simulink model "Three_VSC_Microgrid_Droop_Control"  (R2025a)
settings: Solver=VariableStepAuto  StartTime=0.0  StopTime=10  RelTol=1e-3
InitFcn:
  | fsw=10e3;
  | fref=50;
  | Ts=1/(fsw*fref);
  | Vodref=220*sqrt(2);
  | Voqref=0;
  | Vdc=700;
  | w0=2*pi*fref;
  | 
  | Lf=3.5e-3;
  | Rf=0.1;
  | Cf=50e-6;
  | Lc=0.35e-3;
  | Rc=0.05;
  | 
  | Tci=4/(2*pi*fsw);
  | wci=1/Tci;
  | Kpc=Lf*wci;
  | Kic=Rf*wci;
  | 
  | pm=50;
  | wcv=1/Tci*(1-sind(pm))/(1+sind(pm));
  | wgc=sqrt(wcv*wci);
  | Kpv=Cf*wgc;
  | Kiv=Kpv*wcv;
  | 
  | mp=5e-5;
  | np=3e-3;
libraries: spsThreePhaseSeriesRLCBranchLib x12, slpidlib x12, spsabctodq0Lib x9, spsThreePhaseVIMeasurementLib x6, spsThreePhaseSeriesRLCLoadLib x4, spsDCVoltageSourceLib x3, spsGroundLib x3, spsPWMGenerator2LevelLib x3, spsUniversalBridgeLib x3, spsdq0toabcLib x3, spsThreePhaseBreakerLib x1, spspowerguiLib x1
(part 1 of 2)
settings Model: Creator=DELL  LastModifiedBy=bhargabgogoi

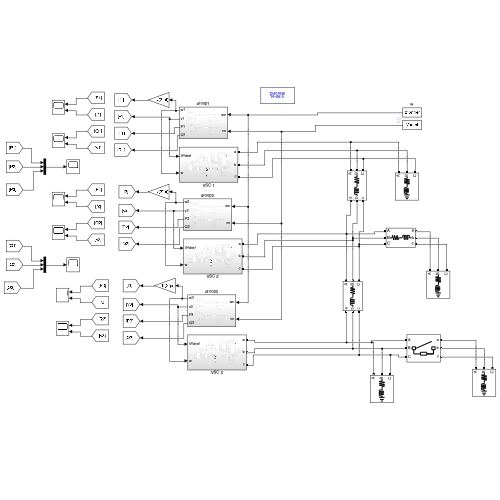
[thumbnail: Simulink's stored preview of the top-level diagram]
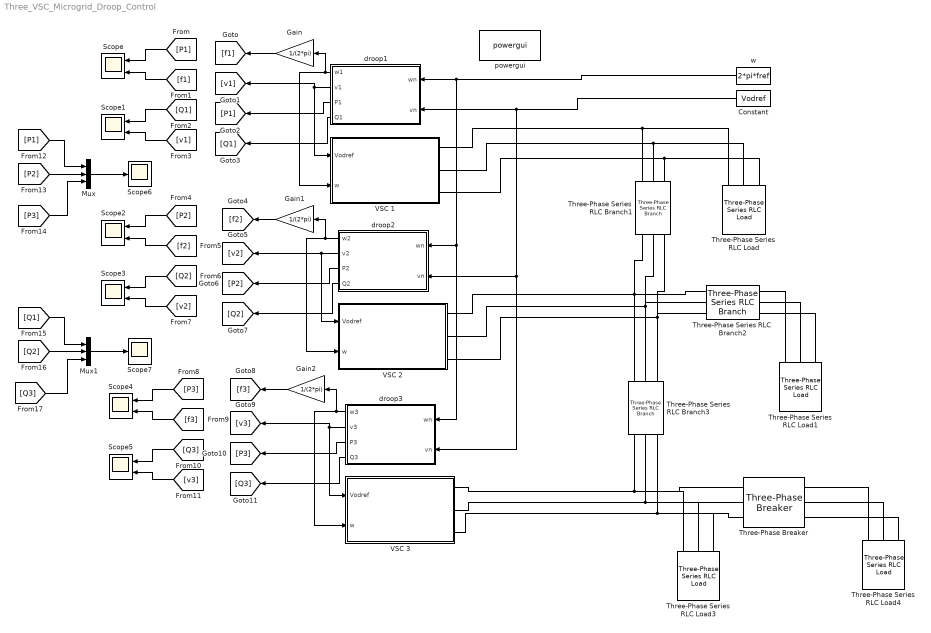
== system Three_VSC_Microgrid_Droop_Control ==
  Constant : Constant  Value=Vodref
  Gain : Gain  Gain=1/(2*pi)
  Gain1 : Gain  Gain=1/(2*pi)
  Gain2 : Gain  Gain=1/(2*pi)
  Mux : Mux  Inputs=3
  Mux1 : Mux  Inputs=3
  Scope{,1..5} (6 alike) : Scope  NumInputPorts=2
      Scope settings: ActiveDisplayYMinimum=-700.9993  ActiveDisplayYMaximum=6308.9933
      Scope1 settings: ActiveDisplayYMinimum=-54.6551  ActiveDisplayYMaximum=491.896  DataLoggingVariableName=ScopeData3
      Scope2 settings: DataLoggingVariableName=ScopeData4
      Scope3 settings: ActiveDisplayYMinimum=-1  ActiveDisplayYMaximum=1  DataLoggingVariableName=ScopeData5
      Scope4 settings: ActiveDisplayYMinimum=-1014.79  ActiveDisplayYMaximum=9133.1097  DataLoggingVariableName=ScopeData6
      Scope5 settings: ActiveDisplayYMinimum=-199.2261  ActiveDisplayYMaximum=1793.0349  DataLoggingVariableName=ScopeData7
  Scope6 : Scope
      settings: ActiveDisplayYMinimum=-1014.79  ActiveDisplayYMaximum=9133.1097  DataLoggingVariableName=ScopeData8
  Scope7 : Scope
      settings: ActiveDisplayYMinimum=-117579.8435  ActiveDisplayYMaximum=146200.4643  DataLoggingVariableName=ScopeData9
  Three-Phase Series RLC Branch1 : spsThreePhaseSeriesRLCBranchLib/Three-Phase Series RLC Branch  LConnTagsString=A|B|C  RConnTagsString=A|B|C  BranchType=RL  Resistance=0.15  Inductance=0.11  Capacitance=1e-6  Measurements=None
  Three-Phase Series RLC Branch2 : spsThreePhaseSeriesRLCBranchLib/Three-Phase Series RLC Branch  LConnTagsString=A|B|C  RConnTagsString=A|B|C  BranchType=RL  Resistance=0.08  Inductance=0.31  Capacitance=1e-6  Measurements=None
  Three-Phase Series RLC Branch3 : spsThreePhaseSeriesRLCBranchLib/Three-Phase Series RLC Branch  LConnTagsString=A|B|C  RConnTagsString=A|B|C  BranchType=RL  Resistance=0.15  Inductance=0.11  Capacitance=1e-6  Measurements=None
  Three-Phase Series RLC Load : spsThreePhaseSeriesRLCLoadLib/Three-Phase Series RLC Load  LConnTagsString=A|B|C  Configuration=Y (grounded)  NominalVoltage=380  Vabc=[1e3 1e3 1e3]  Vabcp=[1e3 1e3 1e3]  NominalFrequency=50  UnbalancedPower=off  ActivePower=5.8e3  InductivePower=0.2e3  CapacitivePower=0  Pabc=[10e3 9e3 11e3]  QLabc=[100 90 110]  QCabc=[100 90 110]  Pabcp=[10e3 9e3 11e3]  QLabcp=[100 90 110]  QCabcp=[100 90 110]  Measurements=None  LoadType=constant Z
  Three-Phase Series RLC Load1 : spsThreePhaseSeriesRLCLoadLib/Three-Phase Series RLC Load  LConnTagsString=A|B|C  Configuration=Y (grounded)  NominalVoltage=380  Vabc=[1e3 1e3 1e3]  Vabcp=[1e3 1e3 1e3]  NominalFrequency=50  UnbalancedPower=off  ActivePower=5.8e3  InductivePower=0.2e3  CapacitivePower=0  Pabc=[10e3 9e3 11e3]  QLabc=[100 90 110]  QCabc=[100 90 110]  Pabcp=[10e3 9e3 11e3]  QLabcp=[100 90 110]  QCabcp=[100 90 110]  Measurements=None  LoadType=constant Z
  Three-Phase Series RLC Load3 : spsThreePhaseSeriesRLCLoadLib/Three-Phase Series RLC Load  LConnTagsString=A|B|C  Configuration=Y (grounded)  NominalVoltage=380  Vabc=[1e3 1e3 1e3]  Vabcp=[1e3 1e3 1e3]  NominalFrequency=50  UnbalancedPower=off  ActivePower=2.3e3  InductivePower=0.3e3  CapacitivePower=0  Pabc=[10e3 9e3 11e3]  QLabc=[100 90 110]  QCabc=[100 90 110]  Pabcp=[10e3 9e3 11e3]  QLabcp=[100 90 110]  QCabcp=[100 90 110]  Measurements=None  LoadType=constant Z
  Three-Phase Series RLC Load4 : spsThreePhaseSeriesRLCLoadLib/Three-Phase Series RLC Load  LConnTagsString=A|B|C  Configuration=Y (grounded)  NominalVoltage=380  Vabc=[1e3 1e3 1e3]  Vabcp=[1e3 1e3 1e3]  NominalFrequency=50  UnbalancedPower=off  ActivePower=6.3e3  InductivePower=1e3  CapacitivePower=0  Pabc=[10e3 9e3 11e3]  QLabc=[100 90 110]  QCabc=[100 90 110]  Pabcp=[10e3 9e3 11e3]  QLabcp=[100 90 110]  QCabcp=[100 90 110]  Measurements=None  LoadType=constant Z
  Three-Phase Breaker : spsThreePhaseBreakerLib/Three-Phase Breaker  InitialState=open  SwitchA=on  SwitchB=on  SwitchC=on  SwitchTimes=[0.4]  External=off  BreakerResistance=0.01  SnubberResistance=1e6  SnubberCapacitance=inf  Measurements=None
  VSC 1 : Subsystem
  VSC 2 : Subsystem
  VSC 3 : Subsystem
  droop1 : Subsystem
  droop2 : Subsystem
  droop3 : Subsystem
  powergui : spspowerguiLib/powergui  Priority=1  SimulationMode=Discrete  SampleTime=1e-06  frequency=60  Iterations=50  frequencyindice=0  Pbase=100e6  ErrMax=1e-4  UnitsV=kV  UnitsW=MW  buscounter=0  FunctionMessages=off  echomessages=off  EnableUseOfTLC=off  CurrentSourceSwitches=off  DisableSnubberDevices=off  DisableRonSwitches=off  DisableVfSwitches=off  DisplayEquations=off  AutomaticDiscreteSolvers=off  SolverType=Tustin/Backward Euler (TBE)  Interpol=off  ExternalGateDelay=off  methode=off  Ts=100  x0status=blocks  SPID=on  SwTol=0  HookPort=off  NonlinearTolerance=1e-4  nMaxIteration=100  ContinueOnMaxIteration=off  RestoreLinks=warning  ResistiveCurrentMeasurement=off  Frange=[0:2:500]  Ylog=off  Xlog=on  ShowGrid=off  save=off  variable=ZData  structure=0  ZoomFFT=off  StartTime=0.0  cycles=1  DisplayStyle=1  fundamental=60  FreqAxis=off  MaxFrequency=1000  frequencyindicesteady=1  RmsSteady=1  display=off
  w : Constant  Value=2*pi*fref
  wires:
  droop1/1(w1) -> Gain/1, VSC 1/2(w)
  droop1/2(v1) -> [v1], VSC 1/1(Vodref)
  w/1 -> droop1/1(wn), droop3/1(wn), droop2/1(wn)
  Constant/1 -> droop3/2(vn), droop2/2(vn), droop1/2(vn)
  droop1/3(P1) -> [P1]
  droop1/4(Q1) -> [Q1]
  droop2/3(P2) -> [P2]
  droop2/4(Q2) -> [Q2]
  droop2/2(v2) -> VSC 2/1(Vodref), [v2]
  droop3/3(P3) -> [P3]
  droop3/4(Q3) -> [Q3]
  droop3/2(v3) -> [v3], VSC 3/1(Vodref)
  [P1] -> Scope/1
  [f1] -> Scope/2
  Gain/1 -> [f1]
  Gain1/1 -> [f2]
  droop2/1(w2) -> Gain1/1, VSC 2/2(w)
  Gain2/1 -> [f3]
  droop3/1(w3) -> VSC 3/2(w), Gain2/1
  [v1] -> Scope1/2
  [Q1] -> Scope1/1
  [f2] -> Scope2/2
  [v2] -> Scope3/2
  [Q2] -> Scope3/1
  [P2] -> Scope2/1
  [f3] -> Scope4/2
  [v3] -> Scope5/2
  [Q3] -> Scope5/1
  [P3] -> Scope4/1
  Mux/1 -> Scope6/1
  [P1] -> Mux/1
  [P2] -> Mux/2
  [P3] -> Mux/3
  [Q2] -> Mux1/2
  Mux1/1 -> Scope7/1
  [Q1] -> Mux1/1
  [Q3] -> Mux1/3
  connections:
  Three-Phase Series RLC Branch3/LConn1 -- VSC 2/RConn1 -- Three-Phase Series RLC Branch2/LConn1 -- Three-Phase Series RLC Branch1/RConn1
  Three-Phase Series RLC Branch3/LConn3 -- Three-Phase Series RLC Branch2/LConn3 -- Three-Phase Series RLC Branch1/RConn3 -- VSC 2/RConn3
  Three-Phase Series RLC Branch3/LConn2 -- Three-Phase Series RLC Branch2/LConn2 -- Three-Phase Series RLC Branch1/RConn2 -- VSC 2/RConn2
  Three-Phase Series RLC Branch1/LConn1 -- VSC 1/RConn1 -- Three-Phase Series RLC Load/LConn1
  Three-Phase Series RLC Branch1/LConn2 -- VSC 1/RConn2 -- Three-Phase Series RLC Load/LConn2
  Three-Phase Series RLC Branch1/LConn3 -- VSC 1/RConn3 -- Three-Phase Series RLC Load/LConn3
  Three-Phase Series RLC Branch3/RConn1 -- Three-Phase Series RLC Load3/LConn1 -- Three-Phase Breaker/LConn1 -- VSC 3/RConn1
  Three-Phase Series RLC Branch3/RConn2 -- Three-Phase Series RLC Load3/LConn2 -- Three-Phase Breaker/LConn2 -- VSC 3/RConn2
  Three-Phase Series RLC Branch3/RConn3 -- Three-Phase Breaker/LConn3 -- Three-Phase Series RLC Load3/LConn3 -- VSC 3/RConn3
  Three-Phase Series RLC Branch2/RConn1 -- Three-Phase Series RLC Load1/LConn1
  Three-Phase Series RLC Load1/LConn2 -- Three-Phase Series RLC Branch2/RConn2
  Three-Phase Series RLC Load1/LConn3 -- Three-Phase Series RLC Branch2/RConn3
  Three-Phase Series RLC Load4/LConn1 -- Three-Phase Breaker/RConn1
  Three-Phase Series RLC Load4/LConn2 -- Three-Phase Breaker/RConn2
  Three-Phase Breaker/RConn3 -- Three-Phase Series RLC Load4/LConn3

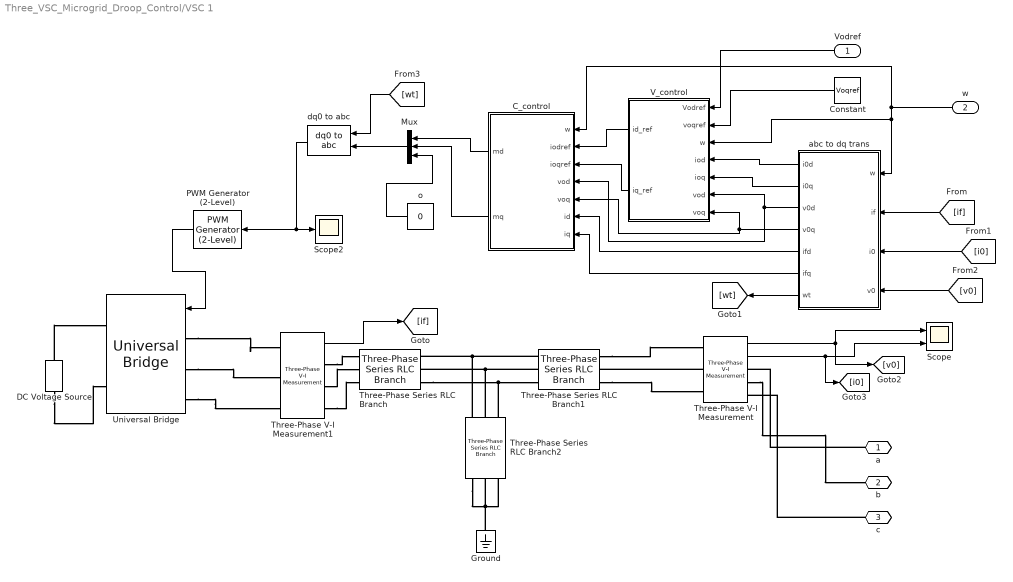
== system Three_VSC_Microgrid_Droop_Control/VSC 1 ==
  Vodref : Inport
  w : Inport  Port=2
  C_control : Subsystem
  Constant : Constant  Value=Voqref
  DC Voltage Source : spsDCVoltageSourceLib/DC Voltage Source  Amplitude=700  Measurements=None
  Ground : spsGroundLib/Ground  LConnTagsString=a
  Mux : Mux  Inputs=3
  PWM Generator (2-Level) : spsPWMGenerator2LevelLib/PWM Generator (2-Level)  ModulatorType=Three-phase bridge (6 pulses)  ModulatorMode=Unsynchronized  Fc=fsw  Pc=90  nF=200  MinMax="[ -1  1 ]"  SamplingTechnique=Natural  ModulatingSignals=off  m=0.8  Freq=60  Phase=0  Ts=0  ShowCarrierOutport=off
  Scope : Scope  NumInputPorts=2
      settings: ActiveDisplayYMinimum=-489.452  ActiveDisplayYMaximum=403.6649
  Scope2 : Scope
      settings: ActiveDisplayYMinimum=-390905.5617  ActiveDisplayYMaximum=341304.2831  DataLoggingVariableName=ScopeData2
  Three-Phase Series RLC Branch : spsThreePhaseSeriesRLCBranchLib/Three-Phase Series RLC Branch  LConnTagsString=A|B|C  RConnTagsString=A|B|C  BranchType=RL  Resistance=Rf  Inductance=Lf  Capacitance=0  Measurements=None
  Three-Phase Series RLC Branch1 : spsThreePhaseSeriesRLCBranchLib/Three-Phase Series RLC Branch  LConnTagsString=A|B|C  RConnTagsString=A|B|C  BranchType=RL  Resistance=Rc  Inductance=Lc  Capacitance=0  Measurements=None
  Three-Phase Series RLC Branch2 : spsThreePhaseSeriesRLCBranchLib/Three-Phase Series RLC Branch  LConnTagsString=A|B|C  RConnTagsString=A|B|C  BranchType=C  Resistance=Rf  Inductance=Lf  Capacitance=Cf  Measurements=None
  Three-Phase V-I Measurement : spsThreePhaseVIMeasurementLib/Three-Phase V-I Measurement  VoltageMeasurement=phase-to-ground  SetLabelV=off  LabelV=Vabc  Vpu=off  VpuLL=off  CurrentMeasurement=yes  SetLabelI=off  LabelI=Iabc  Ipu=off  Pbase=100e6  Vbase=500e3  OutputType=Complex  PhasorSimulation=off  PSBequivalent=0
  Three-Phase V-I Measurement1 : spsThreePhaseVIMeasurementLib/Three-Phase V-I Measurement  VoltageMeasurement=no  SetLabelV=off  LabelV=Vabc  Vpu=off  VpuLL=off  CurrentMeasurement=yes  SetLabelI=off  LabelI=Iabc  Ipu=off  Pbase=100e6  Vbase=500e3  OutputType=Complex  PhasorSimulation=off  PSBequivalent=0
  Universal Bridge : spsUniversalBridgeLib/Universal Bridge  Arms=3  SnubberResistance=1e5  SnubberCapacitance=inf  Device=IGBT / Diodes  Ron=1e-3  Lon=0  ForwardVoltages="[  0  0  ]"  ForwardVoltage=0  GTOparameters=[ 10e-6 , 20e-6 ]  IGBTparameters=[ 1e-6 , 2e-6 ]  Measurements=None  Measurements_2=None  converterType=Rectifier
  V_control : Subsystem
  abc to dq trans : Subsystem
  dq0 to abc : spsdq0toabcLib/dq0 to abc  Alignment=90 degrees behind phase A axis
  o : Constant  Value=0
  a : PMIOPort  Side=Right
  b : PMIOPort  Port=2  Side=Right
  c : PMIOPort  Port=3  Side=Right
  wires:
  Three-Phase V-I Measurement1/1 -> [if]
  [v0] -> abc to dq trans/4(v0)
  V_control/1(id_ref) -> C_control/2(iodref)
  abc to dq trans/6(ifq) -> C_control/7(iq)
  [wt] -> dq0 to abc/2
  Mux/1 -> dq0 to abc/1
  abc to dq trans/1(i0d) -> V_control/4(iod)
  abc to dq trans/3(v0d) -> V_control/6(vod), C_control/4(vod)
  V_control/2(iq_ref) -> C_control/3(ioqref)
  abc to dq trans/4(v0q) -> V_control/7(voq), C_control/5(voq)
  C_control/1(md) -> Mux/1
  [i0] -> abc to dq trans/3(i0)
  PWM Generator (2-Level)/1 -> Universal Bridge/1
  abc to dq trans/5(ifd) -> C_control/6(id)
  abc to dq trans/2(i0q) -> V_control/5(ioq)
  Three-Phase V-I Measurement/1 -> [v0], Scope/1
  o/1 -> Mux/3
  abc to dq trans/7(wt) -> [wt]
  dq0 to abc/1 -> Scope2/1, PWM Generator (2-Level)/1
  [if] -> abc to dq trans/2(if)
  C_control/2(mq) -> Mux/2
  Three-Phase V-I Measurement/2 -> Scope/2, [i0]
  Constant/1 -> V_control/2(voqref)
  Vodref/1 -> V_control/1(Vodref)
  w/1 -> V_control/3(w), abc to dq trans/1(w), C_control/1(w)
  connections:
  DC Voltage Source/LConn1 -- Universal Bridge/RConn2
  Universal Bridge/LConn3 -- Three-Phase V-I Measurement1/LConn3
  Universal Bridge/LConn2 -- Three-Phase V-I Measurement1/LConn2
  DC Voltage Source/RConn1 -- Universal Bridge/RConn1
  Three-Phase Series RLC Branch/RConn3 -- Three-Phase Series RLC Branch2/LConn3 -- Three-Phase Series RLC Branch1/LConn3
  Three-Phase V-I Measurement1/RConn3 -- Three-Phase Series RLC Branch/LConn3
  Three-Phase V-I Measurement1/RConn1 -- Three-Phase Series RLC Branch/LConn1
  Three-Phase Series RLC Branch1/RConn1 -- Three-Phase V-I Measurement/LConn1
  Universal Bridge/LConn1 -- Three-Phase V-I Measurement1/LConn1
  Three-Phase Series RLC Branch1/LConn1 -- Three-Phase Series RLC Branch/RConn1 -- Three-Phase Series RLC Branch2/LConn1
  c/RConn1 -- Three-Phase V-I Measurement/RConn3
  Three-Phase V-I Measurement1/RConn2 -- Three-Phase Series RLC Branch/LConn2
  Ground/LConn1 -- Three-Phase Series RLC Branch2/RConn2 -- Three-Phase Series RLC Branch2/RConn3 -- Three-Phase Series RLC Branch2/RConn1
  Three-Phase Series RLC Branch1/LConn2 -- Three-Phase Series RLC Branch/RConn2 -- Three-Phase Series RLC Branch2/LConn2
  Three-Phase V-I Measurement/LConn2 -- Three-Phase Series RLC Branch1/RConn2
  Three-Phase Series RLC Branch1/RConn3 -- Three-Phase V-I Measurement/LConn3
  a/RConn1 -- Three-Phase V-I Measurement/RConn1
  Three-Phase V-I Measurement/RConn2 -- b/RConn1

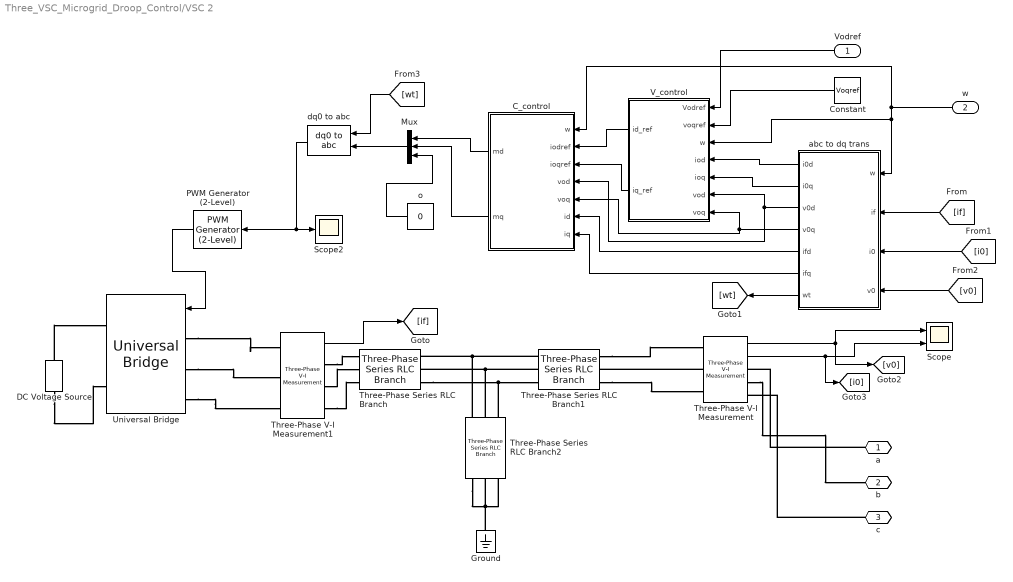
== system Three_VSC_Microgrid_Droop_Control/VSC 2 ==
  Vodref : Inport
  w : Inport  Port=2
  C_control : Subsystem
  Constant : Constant  Value=Voqref
  DC Voltage Source : spsDCVoltageSourceLib/DC Voltage Source  Amplitude=700  Measurements=None
  Ground : spsGroundLib/Ground  LConnTagsString=a
  Mux : Mux  Inputs=3
  PWM Generator (2-Level) : spsPWMGenerator2LevelLib/PWM Generator (2-Level)  ModulatorType=Three-phase bridge (6 pulses)  ModulatorMode=Unsynchronized  Fc=fsw  Pc=90  nF=200  MinMax="[ -1  1 ]"  SamplingTechnique=Natural  ModulatingSignals=off  m=0.8  Freq=60  Phase=0  Ts=0  ShowCarrierOutport=off
  Scope : Scope  NumInputPorts=2
      settings: ActiveDisplayYMinimum=-489.452  ActiveDisplayYMaximum=403.6649
  Scope2 : Scope
      settings: ActiveDisplayYMinimum=-4.1735  ActiveDisplayYMaximum=4.1686  DataLoggingVariableName=ScopeData2
  Three-Phase Series RLC Branch : spsThreePhaseSeriesRLCBranchLib/Three-Phase Series RLC Branch  LConnTagsString=A|B|C  RConnTagsString=A|B|C  BranchType=RL  Resistance=Rf  Inductance=Lf  Capacitance=0  Measurements=None
  Three-Phase Series RLC Branch1 : spsThreePhaseSeriesRLCBranchLib/Three-Phase Series RLC Branch  LConnTagsString=A|B|C  RConnTagsString=A|B|C  BranchType=RL  Resistance=Rc  Inductance=Lc  Capacitance=0  Measurements=None
  Three-Phase Series RLC Branch2 : spsThreePhaseSeriesRLCBranchLib/Three-Phase Series RLC Branch  LConnTagsString=A|B|C  RConnTagsString=A|B|C  BranchType=C  Resistance=Rf  Inductance=Lf  Capacitance=Cf  Measurements=None
  Three-Phase V-I Measurement : spsThreePhaseVIMeasurementLib/Three-Phase V-I Measurement  VoltageMeasurement=phase-to-ground  SetLabelV=off  LabelV=Vabc  Vpu=off  VpuLL=off  CurrentMeasurement=yes  SetLabelI=off  LabelI=Iabc  Ipu=off  Pbase=100e6  Vbase=500e3  OutputType=Complex  PhasorSimulation=off  PSBequivalent=0
  Three-Phase V-I Measurement1 : spsThreePhaseVIMeasurementLib/Three-Phase V-I Measurement  VoltageMeasurement=no  SetLabelV=off  LabelV=Vabc  Vpu=off  VpuLL=off  CurrentMeasurement=yes  SetLabelI=off  LabelI=Iabc  Ipu=off  Pbase=100e6  Vbase=500e3  OutputType=Complex  PhasorSimulation=off  PSBequivalent=0
  Universal Bridge : spsUniversalBridgeLib/Universal Bridge  Arms=3  SnubberResistance=1e5  SnubberCapacitance=inf  Device=IGBT / Diodes  Ron=1e-3  Lon=0  ForwardVoltages="[  0  0  ]"  ForwardVoltage=0  GTOparameters=[ 10e-6 , 20e-6 ]  IGBTparameters=[ 1e-6 , 2e-6 ]  Measurements=None  Measurements_2=None  converterType=Rectifier
  V_control : Subsystem
  abc to dq trans : Subsystem
  dq0 to abc : spsdq0toabcLib/dq0 to abc  Alignment=90 degrees behind phase A axis
  o : Constant  Value=0
  a : PMIOPort  Side=Right
  b : PMIOPort  Port=2  Side=Right
  c : PMIOPort  Port=3  Side=Right
  wires:
  Three-Phase V-I Measurement1/1 -> [if]
  [v0] -> abc to dq trans/4(v0)
  V_control/1(id_ref) -> C_control/2(iodref)
  abc to dq trans/6(ifq) -> C_control/7(iq)
  [wt] -> dq0 to abc/2
  Mux/1 -> dq0 to abc/1
  abc to dq trans/1(i0d) -> V_control/4(iod)
  abc to dq trans/3(v0d) -> V_control/6(vod), C_control/4(vod)
  V_control/2(iq_ref) -> C_control/3(ioqref)
  abc to dq trans/4(v0q) -> V_control/7(voq), C_control/5(voq)
  C_control/1(md) -> Mux/1
  [i0] -> abc to dq trans/3(i0)
  PWM Generator (2-Level)/1 -> Universal Bridge/1
  abc to dq trans/5(ifd) -> C_control/6(id)
  abc to dq trans/2(i0q) -> V_control/5(ioq)
  Three-Phase V-I Measurement/1 -> [v0], Scope/1
  o/1 -> Mux/3
  abc to dq trans/7(wt) -> [wt]
  dq0 to abc/1 -> Scope2/1, PWM Generator (2-Level)/1
  [if] -> abc to dq trans/2(if)
  C_control/2(mq) -> Mux/2
  Three-Phase V-I Measurement/2 -> Scope/2, [i0]
  Constant/1 -> V_control/2(voqref)
  Vodref/1 -> V_control/1(Vodref)
  w/1 -> V_control/3(w), abc to dq trans/1(w), C_control/1(w)
  connections:
  DC Voltage Source/LConn1 -- Universal Bridge/RConn2
  Universal Bridge/LConn3 -- Three-Phase V-I Measurement1/LConn3
  Universal Bridge/LConn2 -- Three-Phase V-I Measurement1/LConn2
  DC Voltage Source/RConn1 -- Universal Bridge/RConn1
  Three-Phase Series RLC Branch/RConn3 -- Three-Phase Series RLC Branch2/LConn3 -- Three-Phase Series RLC Branch1/LConn3
  Three-Phase V-I Measurement1/RConn3 -- Three-Phase Series RLC Branch/LConn3
  Three-Phase V-I Measurement1/RConn1 -- Three-Phase Series RLC Branch/LConn1
  Three-Phase Series RLC Branch1/RConn1 -- Three-Phase V-I Measurement/LConn1
  Universal Bridge/LConn1 -- Three-Phase V-I Measurement1/LConn1
  Three-Phase Series RLC Branch1/LConn1 -- Three-Phase Series RLC Branch/RConn1 -- Three-Phase Series RLC Branch2/LConn1
  c/RConn1 -- Three-Phase V-I Measurement/RConn3
  Three-Phase V-I Measurement1/RConn2 -- Three-Phase Series RLC Branch/LConn2
  Ground/LConn1 -- Three-Phase Series RLC Branch2/RConn2 -- Three-Phase Series RLC Branch2/RConn3 -- Three-Phase Series RLC Branch2/RConn1
  Three-Phase Series RLC Branch1/LConn2 -- Three-Phase Series RLC Branch/RConn2 -- Three-Phase Series RLC Branch2/LConn2
  Three-Phase V-I Measurement/LConn2 -- Three-Phase Series RLC Branch1/RConn2
  Three-Phase Series RLC Branch1/RConn3 -- Three-Phase V-I Measurement/LConn3
  a/RConn1 -- Three-Phase V-I Measurement/RConn1
  Three-Phase V-I Measurement/RConn2 -- b/RConn1

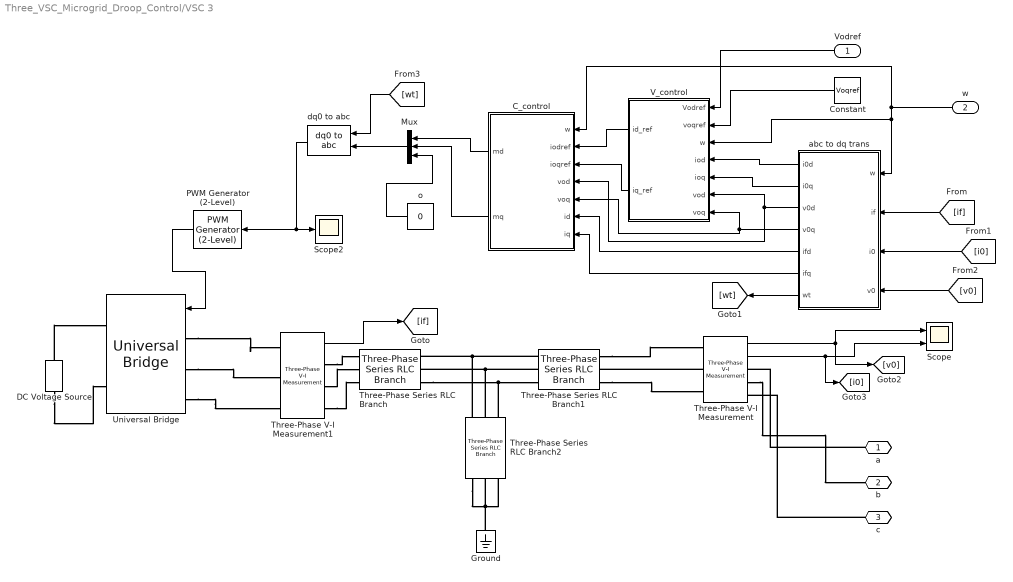
== system Three_VSC_Microgrid_Droop_Control/VSC 3 ==
  Vodref : Inport
  w : Inport  Port=2
  C_control : Subsystem
  Constant : Constant  Value=Voqref
  DC Voltage Source : spsDCVoltageSourceLib/DC Voltage Source  Amplitude=700  Measurements=None
  Ground : spsGroundLib/Ground  LConnTagsString=a
  Mux : Mux  Inputs=3
  PWM Generator (2-Level) : spsPWMGenerator2LevelLib/PWM Generator (2-Level)  ModulatorType=Three-phase bridge (6 pulses)  ModulatorMode=Unsynchronized  Fc=fsw  Pc=90  nF=200  MinMax="[ -1  1 ]"  SamplingTechnique=Natural  ModulatingSignals=off  m=0.8  Freq=60  Phase=0  Ts=0  ShowCarrierOutport=off
  Scope : Scope  NumInputPorts=2
      settings: ActiveDisplayYMinimum=-489.452  ActiveDisplayYMaximum=403.6649
  Scope2 : Scope
      settings: ActiveDisplayYMinimum=-4.1735  ActiveDisplayYMaximum=4.1686  DataLoggingVariableName=ScopeData2
  Three-Phase Series RLC Branch : spsThreePhaseSeriesRLCBranchLib/Three-Phase Series RLC Branch  LConnTagsString=A|B|C  RConnTagsString=A|B|C  BranchType=RL  Resistance=Rf  Inductance=Lf  Capacitance=0  Measurements=None
  Three-Phase Series RLC Branch1 : spsThreePhaseSeriesRLCBranchLib/Three-Phase Series RLC Branch  LConnTagsString=A|B|C  RConnTagsString=A|B|C  BranchType=RL  Resistance=Rc  Inductance=Lc  Capacitance=0  Measurements=None
  Three-Phase Series RLC Branch2 : spsThreePhaseSeriesRLCBranchLib/Three-Phase Series RLC Branch  LConnTagsString=A|B|C  RConnTagsString=A|B|C  BranchType=C  Resistance=Rf  Inductance=Lf  Capacitance=Cf  Measurements=None
  Three-Phase V-I Measurement : spsThreePhaseVIMeasurementLib/Three-Phase V-I Measurement  VoltageMeasurement=phase-to-ground  SetLabelV=off  LabelV=Vabc  Vpu=off  VpuLL=off  CurrentMeasurement=yes  SetLabelI=off  LabelI=Iabc  Ipu=off  Pbase=100e6  Vbase=500e3  OutputType=Complex  PhasorSimulation=off  PSBequivalent=0
  Three-Phase V-I Measurement1 : spsThreePhaseVIMeasurementLib/Three-Phase V-I Measurement  VoltageMeasurement=no  SetLabelV=off  LabelV=Vabc  Vpu=off  VpuLL=off  CurrentMeasurement=yes  SetLabelI=off  LabelI=Iabc  Ipu=off  Pbase=100e6  Vbase=500e3  OutputType=Complex  PhasorSimulation=off  PSBequivalent=0
  Universal Bridge : spsUniversalBridgeLib/Universal Bridge  Arms=3  SnubberResistance=1e5  SnubberCapacitance=inf  Device=IGBT / Diodes  Ron=1e-3  Lon=0  ForwardVoltages="[  0  0  ]"  ForwardVoltage=0  GTOparameters=[ 10e-6 , 20e-6 ]  IGBTparameters=[ 1e-6 , 2e-6 ]  Measurements=None  Measurements_2=None  converterType=Rectifier
  V_control : Subsystem
  abc to dq trans : Subsystem
  dq0 to abc : spsdq0toabcLib/dq0 to abc  Alignment=90 degrees behind phase A axis
  o : Constant  Value=0
  a : PMIOPort  Side=Right
  b : PMIOPort  Port=2  Side=Right
  c : PMIOPort  Port=3  Side=Right
  wires:
  Three-Phase V-I Measurement1/1 -> [if]
  [v0] -> abc to dq trans/4(v0)
  V_control/1(id_ref) -> C_control/2(iodref)
  abc to dq trans/6(ifq) -> C_control/7(iq)
  [wt] -> dq0 to abc/2
  Mux/1 -> dq0 to abc/1
  abc to dq trans/1(i0d) -> V_control/4(iod)
  abc to dq trans/3(v0d) -> V_control/6(vod), C_control/4(vod)
  V_control/2(iq_ref) -> C_control/3(ioqref)
  abc to dq trans/4(v0q) -> V_control/7(voq), C_control/5(voq)
  C_control/1(md) -> Mux/1
  [i0] -> abc to dq trans/3(i0)
  PWM Generator (2-Level)/1 -> Universal Bridge/1
  abc to dq trans/5(ifd) -> C_control/6(id)
  abc to dq trans/2(i0q) -> V_control/5(ioq)
  Three-Phase V-I Measurement/1 -> [v0], Scope/1
  o/1 -> Mux/3
  abc to dq trans/7(wt) -> [wt]
  dq0 to abc/1 -> Scope2/1, PWM Generator (2-Level)/1
  [if] -> abc to dq trans/2(if)
  C_control/2(mq) -> Mux/2
  Three-Phase V-I Measurement/2 -> Scope/2, [i0]
  Constant/1 -> V_control/2(voqref)
  Vodref/1 -> V_control/1(Vodref)
  w/1 -> V_control/3(w), abc to dq trans/1(w), C_control/1(w)
  connections:
  DC Voltage Source/LConn1 -- Universal Bridge/RConn2
  Universal Bridge/LConn3 -- Three-Phase V-I Measurement1/LConn3
  Universal Bridge/LConn2 -- Three-Phase V-I Measurement1/LConn2
  DC Voltage Source/RConn1 -- Universal Bridge/RConn1
  Three-Phase Series RLC Branch/RConn3 -- Three-Phase Series RLC Branch2/LConn3 -- Three-Phase Series RLC Branch1/LConn3
  Three-Phase V-I Measurement1/RConn3 -- Three-Phase Series RLC Branch/LConn3
  Three-Phase V-I Measurement1/RConn1 -- Three-Phase Series RLC Branch/LConn1
  Three-Phase Series RLC Branch1/RConn1 -- Three-Phase V-I Measurement/LConn1
  Universal Bridge/LConn1 -- Three-Phase V-I Measurement1/LConn1
  Three-Phase Series RLC Branch1/LConn1 -- Three-Phase Series RLC Branch/RConn1 -- Three-Phase Series RLC Branch2/LConn1
  c/RConn1 -- Three-Phase V-I Measurement/RConn3
  Three-Phase V-I Measurement1/RConn2 -- Three-Phase Series RLC Branch/LConn2
  Ground/LConn1 -- Three-Phase Series RLC Branch2/RConn2 -- Three-Phase Series RLC Branch2/RConn3 -- Three-Phase Series RLC Branch2/RConn1
  Three-Phase Series RLC Branch1/LConn2 -- Three-Phase Series RLC Branch/RConn2 -- Three-Phase Series RLC Branch2/LConn2
  Three-Phase V-I Measurement/LConn2 -- Three-Phase Series RLC Branch1/RConn2
  Three-Phase Series RLC Branch1/RConn3 -- Three-Phase V-I Measurement/LConn3
  a/RConn1 -- Three-Phase V-I Measurement/RConn1
  Three-Phase V-I Measurement/RConn2 -- b/RConn1

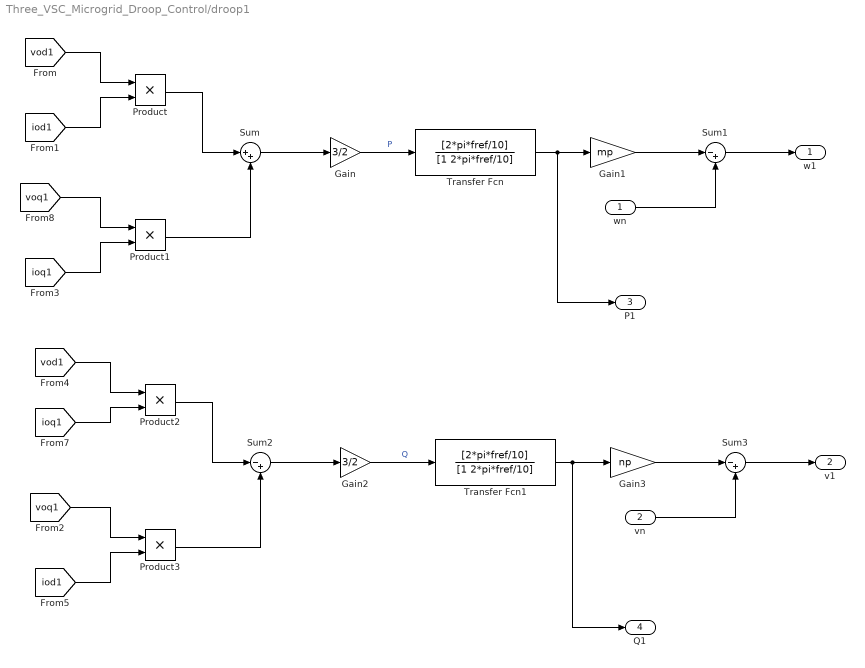
== system Three_VSC_Microgrid_Droop_Control/droop1 ==
  wn : Inport
  vn : Inport  Port=2
  Gain : Gain  Gain=3/2
  Gain1 : Gain  Gain=mp
  Gain2 : Gain  Gain=3/2
  Gain3 : Gain  Gain=np
  Product{,1..3} (4 alike) : Product
  Sum : Sum  Inputs=|++
  Sum1 : Sum  Inputs=|-+
  Sum2 : Sum  Inputs=|-+
  Sum3 : Sum  Inputs=|-+
  Transfer Fcn : TransferFcn  Numerator=[2*pi*fref/10]  Denominator=[1 2*pi*fref/10]
  Transfer Fcn1 : TransferFcn  Numerator=[2*pi*fref/10]  Denominator=[1 2*pi*fref/10]
  w1 : Outport
  v1 : Outport  Port=2
  P1 : Outport  Port=3
  Q1 : Outport  Port=4
  wires:
  Sum3/1 -> v1/1
  Sum1/1 -> w1/1
  [iod1] -> Product3/2
  [ioq1] -> Product2/2
  Sum2/1 -> Gain2/1
  vn/1 -> Sum3/2
  Gain2/1 -> Transfer Fcn1/1  "Q"
  [vod1] -> Product2/1
  Product2/1 -> Sum2/1
  Gain3/1 -> Sum3/1
  Product3/1 -> Sum2/2
  Transfer Fcn1/1 -> Q1/1, Gain3/1
  [voq1] -> Product3/1
  wn/1 -> Sum1/2
  Gain1/1 -> Sum1/1
  Transfer Fcn/1 -> P1/1, Gain1/1
  Gain/1 -> Transfer Fcn/1  "P"
  Sum/1 -> Gain/1
  Product1/1 -> Sum/2
  Product/1 -> Sum/1
  [ioq1] -> Product1/2
  [voq1] -> Product1/1
  [iod1] -> Product/2
  [vod1] -> Product/1

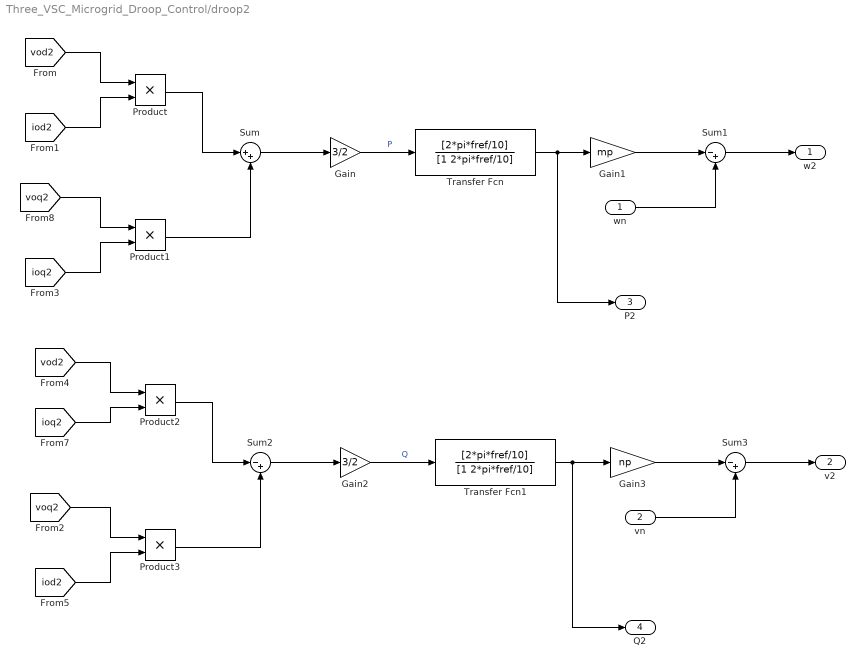
== system Three_VSC_Microgrid_Droop_Control/droop2 ==
  wn : Inport
  vn : Inport  Port=2
  Gain : Gain  Gain=3/2
  Gain1 : Gain  Gain=mp
  Gain2 : Gain  Gain=3/2
  Gain3 : Gain  Gain=np
  Product{,1..3} (4 alike) : Product
  Sum : Sum  Inputs=|++
  Sum1 : Sum  Inputs=|-+
  Sum2 : Sum  Inputs=|-+
  Sum3 : Sum  Inputs=|-+
  Transfer Fcn : TransferFcn  Numerator=[2*pi*fref/10]  Denominator=[1 2*pi*fref/10]
  Transfer Fcn1 : TransferFcn  Numerator=[2*pi*fref/10]  Denominator=[1 2*pi*fref/10]
  w2 : Outport
  v2 : Outport  Port=2
  P2 : Outport  Port=3
  Q2 : Outport  Port=4
  wires:
  Sum3/1 -> v2/1
  Sum1/1 -> w2/1
  [iod2] -> Product3/2
  [ioq2] -> Product2/2
  Sum2/1 -> Gain2/1
  vn/1 -> Sum3/2
  Gain2/1 -> Transfer Fcn1/1  "Q"
  [vod2] -> Product2/1
  Product2/1 -> Sum2/1
  Gain3/1 -> Sum3/1
  Product3/1 -> Sum2/2
  Transfer Fcn1/1 -> Q2/1, Gain3/1
  [voq2] -> Product3/1
  wn/1 -> Sum1/2
  Gain1/1 -> Sum1/1
  Transfer Fcn/1 -> P2/1, Gain1/1
  Gain/1 -> Transfer Fcn/1  "P"
  Sum/1 -> Gain/1
  Product1/1 -> Sum/2
  Product/1 -> Sum/1
  [ioq2] -> Product1/2
  [voq2] -> Product1/1
  [iod2] -> Product/2
  [vod2] -> Product/1

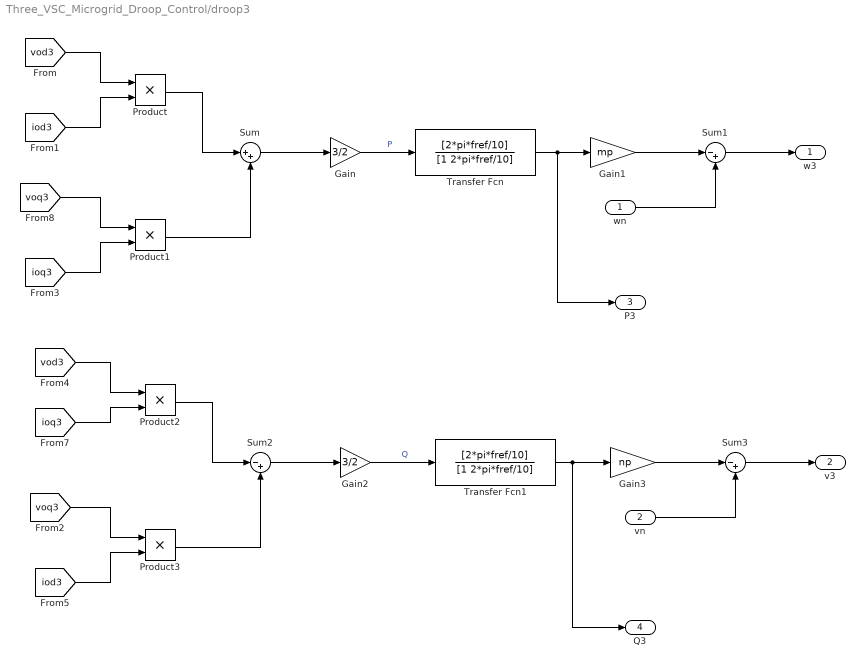
== system Three_VSC_Microgrid_Droop_Control/droop3 ==
  wn : Inport
  vn : Inport  Port=2
  Gain : Gain  Gain=3/2
  Gain1 : Gain  Gain=mp
  Gain2 : Gain  Gain=3/2
  Gain3 : Gain  Gain=np
  Product{,1..3} (4 alike) : Product
  Sum : Sum  Inputs=|++
  Sum1 : Sum  Inputs=|-+
  Sum2 : Sum  Inputs=|-+
  Sum3 : Sum  Inputs=|-+
  Transfer Fcn : TransferFcn  Numerator=[2*pi*fref/10]  Denominator=[1 2*pi*fref/10]
  Transfer Fcn1 : TransferFcn  Numerator=[2*pi*fref/10]  Denominator=[1 2*pi*fref/10]
  w3 : Outport
  v3 : Outport  Port=2
  P3 : Outport  Port=3
  Q3 : Outport  Port=4
  wires:
  Sum3/1 -> v3/1
  Sum1/1 -> w3/1
  [iod3] -> Product3/2
  [ioq3] -> Product2/2
  Sum2/1 -> Gain2/1
  vn/1 -> Sum3/2
  Gain2/1 -> Transfer Fcn1/1  "Q"
  [vod3] -> Product2/1
  Product2/1 -> Sum2/1
  Gain3/1 -> Sum3/1
  Product3/1 -> Sum2/2
  Transfer Fcn1/1 -> Q3/1, Gain3/1
  [voq3] -> Product3/1
  wn/1 -> Sum1/2
  Gain1/1 -> Sum1/1
  Transfer Fcn/1 -> P3/1, Gain1/1
  Gain/1 -> Transfer Fcn/1  "P"
  Sum/1 -> Gain/1
  Product1/1 -> Sum/2
  Product/1 -> Sum/1
  [ioq3] -> Product1/2
  [voq3] -> Product1/1
  [iod3] -> Product/2
  [vod3] -> Product/1

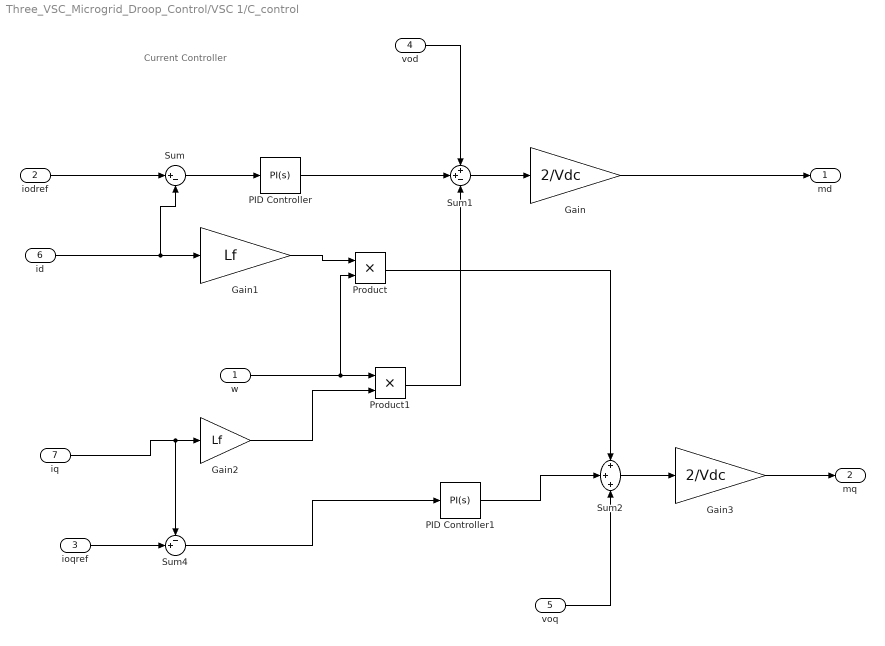
== system Three_VSC_Microgrid_Droop_Control/VSC 1/C_control ==
  note: Current Controller
  w : Inport
  iodref : Inport  Port=2
  ioqref : Inport  Port=3
  vod : Inport  Port=4
  voq : Inport  Port=5
  id : Inport  Port=6
  iq : Inport  Port=7
  Gain : Gain  Gain=2/Vdc
  Gain1 : Gain  Gain=Lf
  Gain2 : Gain  Gain=Lf
  Gain3 : Gain  Gain=2/Vdc
  PID Controller : slpidlib/PID Controller  Controller=PI  Form=Parallel  TimeDomain=Continuous-time  UseExternalTs=off  SampleTime=-1  IntegratorMethod=Forward Euler  FilterMethod=Forward Euler  ControllerParametersSource=internal  P=Kpc  I=Kic  UseKiTs=off  D=0  UseExternalDerivativeSource=off  N=100  UseFilter=on  TunerSelectOption=Transfer Function Based (PID Tuner App)  InitialConditionSource=internal  InitialConditionForIntegrator=0  InitialConditionForFilter=0  DifferentiatorICPrevScaledInput=0  ExternalReset=none  TrackingMode=off  Kt=1  LimitOutput=off  SatLimitsSource=internal  UpperSaturationLimit=inf  LowerSaturationLimit=-inf  LinearizeAsGain=on  AntiWindupMode=none  Kb=1  LimitIntegrator=off  UpperIntegratorSaturationLimit=inf  LowerIntegratorSaturationLimit=-inf  POutMin=[]  POutMax=[]  IOutMin=[]  IOutMax=[]  DOutMin=[]  DOutMax=[]  NOutMin=[]  NOutMax=[]  SumOutMin=[]  SumOutMax=[]  SaturationOutMin=[]  SaturationOutMax=[]  PParamMin=[]  PParamMax=[]  IParamMin=[]  IParamMax=[]  DParamMin=[]  DParamMax=[]  NParamMin=[]  NParamMax=[]  KbParamMin=[]  KbParamMax=[]  KtParamMin=[]  KtParamMax=[]  KbOutMin=[]  KbOutMax=[]  KtOutMin=[]  KtOutMax=[]  IntegratorOutMin=[]  IntegratorOutMax=[]  FilterOutMin=[]  FilterOutMax=[]  SumI1OutMin=[]  SumI1OutMax=[]  SumI2OutMin=[]  SumI2OutMax=[]  SumI3OutMin=[]  SumI3OutMax=[]  SumI4OutMin=[]  SumI4OutMax=[]  SumDOutMin=[]  SumDOutMax=[]  DifferentiatorOutMin=[]  DifferentiatorOutMax=[]  FilterDiffOutCoefMin=[]  FilterDiffOutCoefMax=[]  ReciprocalOutMin=[]  ReciprocalOutMax=[]  SumDenOutMin=[]  SumDenOutMax=[]  SumNumOutMin=[]  SumNumOutMax=[]  DivideOutMin=[]  DivideOutMax=[]  UdiffTsProdOutMin=[]  UdiffTsProdOutMax=[]  NTsProdOutMin=[]  NTsProdOutMax=[]  UintegralTsProdOutMin=[]  UintegralTsProdOutMax=[]  UngainTsProdOutMin=[]  UngainTsProdOutMax=[]  ClampingZeroOutDataTypeStr=Inherit: Inherit via back propagation  ClampingZeroOutMin=[]  ClampingZeroOutMax=[]  FilterDenConstantOutDataTypeStr=Inherit: Inherit via back propagation  FilterDenConstantOutMin=[]  FilterDenConstantOutMax=[]  PCopyOutDataTypeStr=Inherit: Inherit via back propagation  PCopyOutMin=[]  PCopyOutMax=[]  NCopyOutDataTypeStr=Inherit: Inherit via back propagation  NCopyOutMin=[]  NCopyOutMax=[]  IntegratorContinuousStateAttributes=''  IntegratorStateMustResolveToSignalObject=off  IntegratorRTWStateStorageClass=Auto  FilterContinuousStateAttributes=''  FilterStateMustResolveToSignalObject=off  FilterRTWStateStorageClass=Auto  ParallelPVariant=InternalParameters  IdealPVariant=Disabled  IVariant=InternalParameters  DVariant=Disabled  IntegratorVariant=Continuous  SatVariant=Disabled  AWVariant=Passthrough  PCopyVariant=Disabled  TRVariant=Disabled  FdbkBlocksVariant=Forward  IdealPFdbkVariant=Disabled  SatFdbkVariant=Disabled  DerivativeFilterVariant=Disabled  NVariant=Disabled  NCopyVariant=Disabled_SignalSpec  FilterICVariant=Disabled  IntegratorICVariant=InternalICs  ExternalResetVariant=Disabled  TRSumVariant=Passthrough  SumFdbkVariant=Disabled  SumVariant=Sum_PI  TsampFilterVariant=InternalTs  TsampNgainVariant=Passthrough  TsampIntegralVariant=Disabled_SignalSpec  ExternalSaturationOutDataTypeStr=Inherit: Same as second input  DerivativeSourceVariant=Disabled  PreIntVariant=InternalPreInt
  PID Controller1 : slpidlib/PID Controller  Controller=PI  Form=Parallel  TimeDomain=Continuous-time  UseExternalTs=off  SampleTime=-1  IntegratorMethod=Forward Euler  FilterMethod=Forward Euler  ControllerParametersSource=internal  P=Kpc  I=Kic  UseKiTs=off  D=0  UseExternalDerivativeSource=off  N=100  UseFilter=on  TunerSelectOption=Transfer Function Based (PID Tuner App)  InitialConditionSource=internal  InitialConditionForIntegrator=0  InitialConditionForFilter=0  DifferentiatorICPrevScaledInput=0  ExternalReset=none  TrackingMode=off  Kt=1  LimitOutput=off  SatLimitsSource=internal  UpperSaturationLimit=inf  LowerSaturationLimit=-inf  LinearizeAsGain=on  AntiWindupMode=none  Kb=1  LimitIntegrator=off  UpperIntegratorSaturationLimit=inf  LowerIntegratorSaturationLimit=-inf  POutMin=[]  POutMax=[]  IOutMin=[]  IOutMax=[]  DOutMin=[]  DOutMax=[]  NOutMin=[]  NOutMax=[]  SumOutMin=[]  SumOutMax=[]  SaturationOutMin=[]  SaturationOutMax=[]  PParamMin=[]  PParamMax=[]  IParamMin=[]  IParamMax=[]  DParamMin=[]  DParamMax=[]  NParamMin=[]  NParamMax=[]  KbParamMin=[]  KbParamMax=[]  KtParamMin=[]  KtParamMax=[]  KbOutMin=[]  KbOutMax=[]  KtOutMin=[]  KtOutMax=[]  IntegratorOutMin=[]  IntegratorOutMax=[]  FilterOutMin=[]  FilterOutMax=[]  SumI1OutMin=[]  SumI1OutMax=[]  SumI2OutMin=[]  SumI2OutMax=[]  SumI3OutMin=[]  SumI3OutMax=[]  SumI4OutMin=[]  SumI4OutMax=[]  SumDOutMin=[]  SumDOutMax=[]  DifferentiatorOutMin=[]  DifferentiatorOutMax=[]  FilterDiffOutCoefMin=[]  FilterDiffOutCoefMax=[]  ReciprocalOutMin=[]  ReciprocalOutMax=[]  SumDenOutMin=[]  SumDenOutMax=[]  SumNumOutMin=[]  SumNumOutMax=[]  DivideOutMin=[]  DivideOutMax=[]  UdiffTsProdOutMin=[]  UdiffTsProdOutMax=[]  NTsProdOutMin=[]  NTsProdOutMax=[]  UintegralTsProdOutMin=[]  UintegralTsProdOutMax=[]  UngainTsProdOutMin=[]  UngainTsProdOutMax=[]  ClampingZeroOutDataTypeStr=Inherit: Inherit via back propagation  ClampingZeroOutMin=[]  ClampingZeroOutMax=[]  FilterDenConstantOutDataTypeStr=Inherit: Inherit via back propagation  FilterDenConstantOutMin=[]  FilterDenConstantOutMax=[]  PCopyOutDataTypeStr=Inherit: Inherit via back propagation  PCopyOutMin=[]  PCopyOutMax=[]  NCopyOutDataTypeStr=Inherit: Inherit via back propagation  NCopyOutMin=[]  NCopyOutMax=[]  IntegratorContinuousStateAttributes=''  IntegratorStateMustResolveToSignalObject=off  IntegratorRTWStateStorageClass=Auto  FilterContinuousStateAttributes=''  FilterStateMustResolveToSignalObject=off  FilterRTWStateStorageClass=Auto  ParallelPVariant=InternalParameters  IdealPVariant=Disabled  IVariant=InternalParameters  DVariant=Disabled  IntegratorVariant=Continuous  SatVariant=Disabled  AWVariant=Passthrough  PCopyVariant=Disabled  TRVariant=Disabled  FdbkBlocksVariant=Forward  IdealPFdbkVariant=Disabled  SatFdbkVariant=Disabled  DerivativeFilterVariant=Disabled  NVariant=Disabled  NCopyVariant=Disabled_SignalSpec  FilterICVariant=Disabled  IntegratorICVariant=InternalICs  ExternalResetVariant=Disabled  TRSumVariant=Passthrough  SumFdbkVariant=Disabled  SumVariant=Sum_PI  TsampFilterVariant=InternalTs  TsampNgainVariant=Passthrough  TsampIntegralVariant=Disabled_SignalSpec  ExternalSaturationOutDataTypeStr=Inherit: Same as second input  DerivativeSourceVariant=Disabled  PreIntVariant=InternalPreInt
  Product : Product
  Product1 : Product
  Sum : Sum  Inputs=|+-
  Sum1 : Sum  Inputs=++-
  Sum2 : Sum  Inputs=+++
  Sum4 : Sum  Inputs=-+|
  md : Outport
  mq : Outport  Port=2
  wires:
  Sum/1 -> PID Controller/1
  iodref/1 -> Sum/1
  PID Controller/1 -> Sum1/2
  vod/1 -> Sum1/1
  Sum1/1 -> Gain/1
  Gain/1 -> md/1
  id/1 -> Sum/2, Gain1/1
  Gain1/1 -> Product/1
  iq/1 -> Sum4/1, Gain2/1
  Gain2/1 -> Product1/2
  Product1/1 -> Sum1/3
  Product/1 -> Sum2/1
  PID Controller1/1 -> Sum2/2
  voq/1 -> Sum2/3
  ioqref/1 -> Sum4/2
  Sum4/1 -> PID Controller1/1
  Sum2/1 -> Gain3/1
  Gain3/1 -> mq/1
  w/1 -> Product/2, Product1/1

== system Three_VSC_Microgrid_Droop_Control/VSC 1/V_control ==
  note: Voltage Controller
  Vodref : Inport
  voqref : Inport  Port=2
  w : Inport  Port=3
  iod : Inport  Port=4
  ioq : Inport  Port=5
  vod : Inport  Port=6
  voq : Inport  Port=7
  Gain : Gain  Gain=Cf
  Gain1 : Gain  Gain=Cf
  PID Controller : slpidlib/PID Controller  Controller=PI  Form=Parallel  TimeDomain=Continuous-time  UseExternalTs=off  SampleTime=-1  IntegratorMethod=Forward Euler  FilterMethod=Forward Euler  ControllerParametersSource=internal  P=Kpv  I=Kiv  UseKiTs=off  D=0  UseExternalDerivativeSource=off  N=100  UseFilter=on  TunerSelectOption=Transfer Function Based (PID Tuner App)  InitialConditionSource=internal  InitialConditionForIntegrator=0  InitialConditionForFilter=0  DifferentiatorICPrevScaledInput=0  ExternalReset=none  TrackingMode=off  Kt=1  LimitOutput=off  SatLimitsSource=internal  UpperSaturationLimit=inf  LowerSaturationLimit=-inf  LinearizeAsGain=on  AntiWindupMode=none  Kb=1  LimitIntegrator=off  UpperIntegratorSaturationLimit=inf  LowerIntegratorSaturationLimit=-inf  POutMin=[]  POutMax=[]  IOutMin=[]  IOutMax=[]  DOutMin=[]  DOutMax=[]  NOutMin=[]  NOutMax=[]  SumOutMin=[]  SumOutMax=[]  SaturationOutMin=[]  SaturationOutMax=[]  PParamMin=[]  PParamMax=[]  IParamMin=[]  IParamMax=[]  DParamMin=[]  DParamMax=[]  NParamMin=[]  NParamMax=[]  KbParamMin=[]  KbParamMax=[]  KtParamMin=[]  KtParamMax=[]  KbOutMin=[]  KbOutMax=[]  KtOutMin=[]  KtOutMax=[]  IntegratorOutMin=[]  IntegratorOutMax=[]  FilterOutMin=[]  FilterOutMax=[]  SumI1OutMin=[]  SumI1OutMax=[]  SumI2OutMin=[]  SumI2OutMax=[]  SumI3OutMin=[]  SumI3OutMax=[]  SumI4OutMin=[]  SumI4OutMax=[]  SumDOutMin=[]  SumDOutMax=[]  DifferentiatorOutMin=[]  DifferentiatorOutMax=[]  FilterDiffOutCoefMin=[]  FilterDiffOutCoefMax=[]  ReciprocalOutMin=[]  ReciprocalOutMax=[]  SumDenOutMin=[]  SumDenOutMax=[]  SumNumOutMin=[]  SumNumOutMax=[]  DivideOutMin=[]  DivideOutMax=[]  UdiffTsProdOutMin=[]  UdiffTsProdOutMax=[]  NTsProdOutMin=[]  NTsProdOutMax=[]  UintegralTsProdOutMin=[]  UintegralTsProdOutMax=[]  UngainTsProdOutMin=[]  UngainTsProdOutMax=[]  ClampingZeroOutDataTypeStr=Inherit: Inherit via back propagation  ClampingZeroOutMin=[]  ClampingZeroOutMax=[]  FilterDenConstantOutDataTypeStr=Inherit: Inherit via back propagation  FilterDenConstantOutMin=[]  FilterDenConstantOutMax=[]  PCopyOutDataTypeStr=Inherit: Inherit via back propagation  PCopyOutMin=[]  PCopyOutMax=[]  NCopyOutDataTypeStr=Inherit: Inherit via back propagation  NCopyOutMin=[]  NCopyOutMax=[]  IntegratorContinuousStateAttributes=''  IntegratorStateMustResolveToSignalObject=off  IntegratorRTWStateStorageClass=Auto  FilterContinuousStateAttributes=''  FilterStateMustResolveToSignalObject=off  FilterRTWStateStorageClass=Auto  ParallelPVariant=InternalParameters  IdealPVariant=Disabled  IVariant=InternalParameters  DVariant=Disabled  IntegratorVariant=Continuous  SatVariant=Disabled  AWVariant=Passthrough  PCopyVariant=Disabled  TRVariant=Disabled  FdbkBlocksVariant=Forward  IdealPFdbkVariant=Disabled  SatFdbkVariant=Disabled  DerivativeFilterVariant=Disabled  NVariant=Disabled  NCopyVariant=Disabled_SignalSpec  FilterICVariant=Disabled  IntegratorICVariant=InternalICs  ExternalResetVariant=Disabled  TRSumVariant=Passthrough  SumFdbkVariant=Disabled  SumVariant=Sum_PI  TsampFilterVariant=InternalTs  TsampNgainVariant=Passthrough  TsampIntegralVariant=Disabled_SignalSpec  ExternalSaturationOutDataTypeStr=Inherit: Same as second input  DerivativeSourceVariant=Disabled  PreIntVariant=InternalPreInt
  PID Controller1 : slpidlib/PID Controller  Controller=PI  Form=Parallel  TimeDomain=Continuous-time  UseExternalTs=off  SampleTime=-1  IntegratorMethod=Forward Euler  FilterMethod=Forward Euler  ControllerParametersSource=internal  P=Kpv  I=Kiv  UseKiTs=off  D=0  UseExternalDerivativeSource=off  N=100  UseFilter=on  TunerSelectOption=Transfer Function Based (PID Tuner App)  InitialConditionSource=internal  InitialConditionForIntegrator=0  InitialConditionForFilter=0  DifferentiatorICPrevScaledInput=0  ExternalReset=none  TrackingMode=off  Kt=1  LimitOutput=off  SatLimitsSource=internal  UpperSaturationLimit=inf  LowerSaturationLimit=-inf  LinearizeAsGain=on  AntiWindupMode=none  Kb=1  LimitIntegrator=off  UpperIntegratorSaturationLimit=inf  LowerIntegratorSaturationLimit=-inf  POutMin=[]  POutMax=[]  IOutMin=[]  IOutMax=[]  DOutMin=[]  DOutMax=[]  NOutMin=[]  NOutMax=[]  SumOutMin=[]  SumOutMax=[]  SaturationOutMin=[]  SaturationOutMax=[]  PParamMin=[]  PParamMax=[]  IParamMin=[]  IParamMax=[]  DParamMin=[]  DParamMax=[]  NParamMin=[]  NParamMax=[]  KbParamMin=[]  KbParamMax=[]  KtParamMin=[]  KtParamMax=[]  KbOutMin=[]  KbOutMax=[]  KtOutMin=[]  KtOutMax=[]  IntegratorOutMin=[]  IntegratorOutMax=[]  FilterOutMin=[]  FilterOutMax=[]  SumI1OutMin=[]  SumI1OutMax=[]  SumI2OutMin=[]  SumI2OutMax=[]  SumI3OutMin=[]  SumI3OutMax=[]  SumI4OutMin=[]  SumI4OutMax=[]  SumDOutMin=[]  SumDOutMax=[]  DifferentiatorOutMin=[]  DifferentiatorOutMax=[]  FilterDiffOutCoefMin=[]  FilterDiffOutCoefMax=[]  ReciprocalOutMin=[]  ReciprocalOutMax=[]  SumDenOutMin=[]  SumDenOutMax=[]  SumNumOutMin=[]  SumNumOutMax=[]  DivideOutMin=[]  DivideOutMax=[]  UdiffTsProdOutMin=[]  UdiffTsProdOutMax=[]  NTsProdOutMin=[]  NTsProdOutMax=[]  UintegralTsProdOutMin=[]  UintegralTsProdOutMax=[]  UngainTsProdOutMin=[]  UngainTsProdOutMax=[]  ClampingZeroOutDataTypeStr=Inherit: Inherit via back propagation  ClampingZeroOutMin=[]  ClampingZeroOutMax=[]  FilterDenConstantOutDataTypeStr=Inherit: Inherit via back propagation  FilterDenConstantOutMin=[]  FilterDenConstantOutMax=[]  PCopyOutDataTypeStr=Inherit: Inherit via back propagation  PCopyOutMin=[]  PCopyOutMax=[]  NCopyOutDataTypeStr=Inherit: Inherit via back propagation  NCopyOutMin=[]  NCopyOutMax=[]  IntegratorContinuousStateAttributes=''  IntegratorStateMustResolveToSignalObject=off  IntegratorRTWStateStorageClass=Auto  FilterContinuousStateAttributes=''  FilterStateMustResolveToSignalObject=off  FilterRTWStateStorageClass=Auto  ParallelPVariant=InternalParameters  IdealPVariant=Disabled  IVariant=InternalParameters  DVariant=Disabled  IntegratorVariant=Continuous  SatVariant=Disabled  AWVariant=Passthrough  PCopyVariant=Disabled  TRVariant=Disabled  FdbkBlocksVariant=Forward  IdealPFdbkVariant=Disabled  SatFdbkVariant=Disabled  DerivativeFilterVariant=Disabled  NVariant=Disabled  NCopyVariant=Disabled_SignalSpec  FilterICVariant=Disabled  IntegratorICVariant=InternalICs  ExternalResetVariant=Disabled  TRSumVariant=Passthrough  SumFdbkVariant=Disabled  SumVariant=Sum_PI  TsampFilterVariant=InternalTs  TsampNgainVariant=Passthrough  TsampIntegralVariant=Disabled_SignalSpec  ExternalSaturationOutDataTypeStr=Inherit: Same as second input  DerivativeSourceVariant=Disabled  PreIntVariant=InternalPreInt
  Product : Product
  Product1 : Product
  Sum : Sum  Inputs=|+-
  Sum1 : Sum  Inputs=++-
  Sum2 : Sum  Inputs=+++
  Sum3 : Sum  Inputs=-+|
  id_ref : Outport
  iq_ref : Outport  Port=2
  wires:
  Vodref/1 -> Sum/1
  Sum/1 -> PID Controller/1
  PID Controller/1 -> Sum1/2
  iod/1 -> Sum1/1
  Sum1/1 -> id_ref/1
  vod/1 -> Sum/2, Gain/1
  Gain/1 -> Product/1
  voq/1 -> Sum3/1, Gain1/1
  Gain1/1 -> Product1/2
  Product1/1 -> Sum1/3
  voqref/1 -> Sum3/2
  Sum3/1 -> PID Controller1/1
  PID Controller1/1 -> Sum2/2
  Product/1 -> Sum2/1
  Sum2/1 -> iq_ref/1
  ioq/1 -> Sum2/3
  w/1 -> Product/2, Product1/1

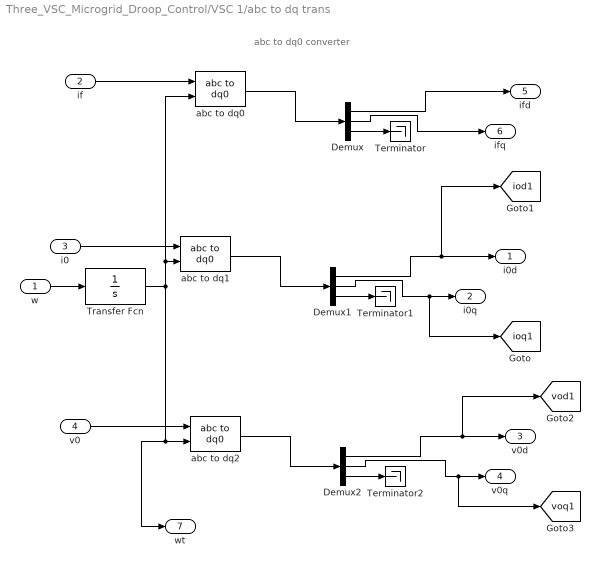
== system Three_VSC_Microgrid_Droop_Control/VSC 1/abc to dq trans ==
  note: abc to dq0 converter
  w : Inport
  if : Inport  Port=2
  i0 : Inport  Port=3
  v0 : Inport  Port=4
  Demux : Demux  Outputs=3
  Demux1 : Demux  Outputs=3
  Demux2 : Demux  Outputs=3
  Terminator : Terminator
  Terminator1 : Terminator
  Terminator2 : Terminator
  Transfer Fcn : TransferFcn  Denominator=[1 0]
  abc to dq0 : spsabctodq0Lib/abc to dq0  Alignment=90 degrees behind phase A axis
  abc to dq1 : spsabctodq0Lib/abc to dq0  Alignment=90 degrees behind phase A axis
  abc to dq2 : spsabctodq0Lib/abc to dq0  Alignment=90 degrees behind phase A axis
  i0d : Outport
  i0q : Outport  Port=2
  v0d : Outport  Port=3
  v0q : Outport  Port=4
  ifd : Outport  Port=5
  ifq : Outport  Port=6
  wt : Outport  Port=7
  tag scope: iod1=global, ioq1=global, vod1=global, voq1=global
  wires:
  if/1 -> abc to dq0/1
  abc to dq0/1 -> Demux/1
  Demux/1 -> ifd/1
  Demux/2 -> ifq/1
  Demux/3 -> Terminator/1
  Demux1/1 -> [iod1], i0d/1
  i0/1 -> abc to dq1/1
  Demux1/2 -> [ioq1], i0q/1
  abc to dq1/1 -> Demux1/1
  Demux1/3 -> Terminator1/1
  Demux2/1 -> [vod1], v0d/1
  v0/1 -> abc to dq2/1
  Demux2/2 -> [voq1], v0q/1
  abc to dq2/1 -> Demux2/1
  Demux2/3 -> Terminator2/1
  w/1 -> Transfer Fcn/1
  Transfer Fcn/1 -> wt/1, abc to dq2/2, abc to dq0/2, abc to dq1/2
